simulink model "LV_Distribution"  (R2026b)
settings: Solver=VariableStepAuto
undefined symbols (not defined in the file or in its folder): P, Ts
libraries: nesl_utility x18, fl_lib x13, ee_lib x8, simulink x5, eeGeneralControl x1
settings Model: Creator=aomar  LastModifiedBy=aomar

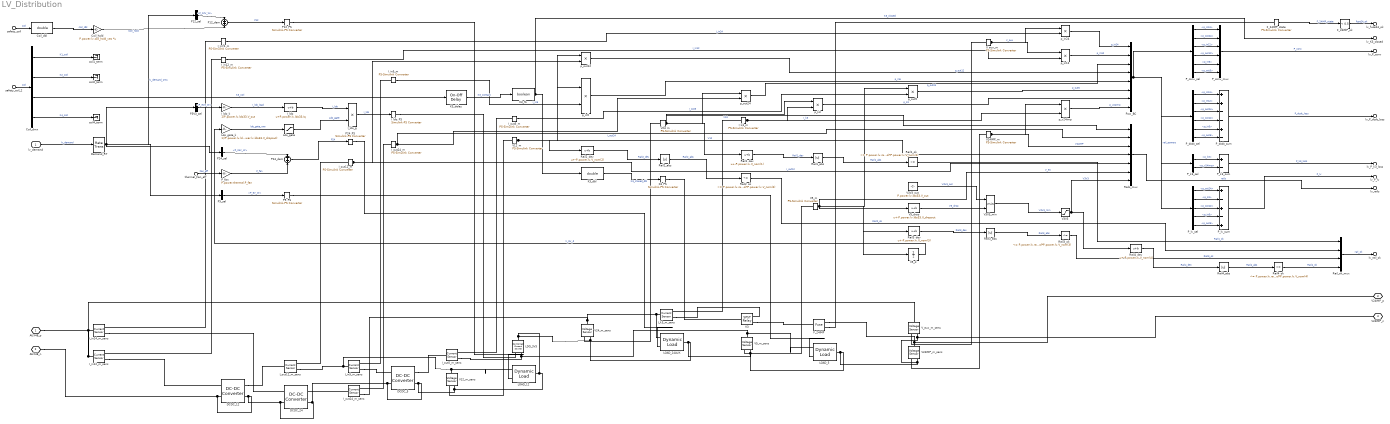
== system LV_Distribution ==
  lv_demand : Inport  OutDataTypeStr=Bus: Bus_LV_LoadDemand  SampleTime=Ts.ctrl
  thermal_Fan_eff : Inport  Port=2  PortName=thermal  Element=Fan_eff
  safety_coil : Inport  Port=3  PortName=safety  Element=coil
  safety_coil_2 : Inport  Port=3  PortName=safety  Element=coil
  Coil_dbl : DataTypeConversion  OutDataTypeStr=double  SaturateOnIntegerOverflow=off  RndMeth=Floor
  Coil_dmx : Demux
  Coil_hold : Gain  Gain=P.power.lv.coil_hold_vec  Multiplication=Matrix(K*u)
  DCDC_12 : ee_lib/Semiconductors & Converters/Converters/DC-DC Converter  Vref_option=ee.enum.converters.voltageref.internal  v_ref=P.power.lv.dcdc12.v_ref V  P_rated=P.power.lv.dcdc12.P_rated W  droop_enabled=false  droop_param=ee.enum.converters.droop.value  droop=0.1 V/A  droop_percent=2  Vref_droop=10 V  reversible=ee.enum.converters.directionality.unidirectional  G_diode=1e-8 1/Ohm  P_fixed=P.power.lv.dcdc12.P_fixed W  losses_option=ee.enum.converters.lossesOption.proportionalToSquaredCurrent  eff_rated=P.power.lv.dcdc12.eff_rated  tableOption=ee.enum.converters.lossTableOptionThermal.currentTemp  i_eff_vec=[-2, -1, 1, 2] A  v_eff_vec=[15, 30, 45] V  eff_vec=[66, 76, 80, 74]  eff_2D_table=[66, 66, 66; 76, 76, 76; 80, 80, 80; 74, 74, 74]  model_dynamics=ee.enum.converters.dynamics.yes  tau=P.power.lv.dcdc12.tau s  v_ini=0 V  v1_min=P.power.lv.dcdc12.v1_min V  R1=P.power.lv.dcdc12.R1 Ohm  R2=P.power.lv.dcdc12.R2 Ohm  T_eff_vec=[280, 300, 320] K  eff_3D_table=repmat([66; 76; 80; 74], 1, 3, 3)  thermal_mass=100 J/K  initial_temperature=298.15 K
  DCDC_24 : ee_lib/Semiconductors & Converters/Converters/DC-DC Converter  Vref_option=ee.enum.converters.voltageref.internal  v_ref=P.power.lv.dcdc24.v_ref V  P_rated=P.power.lv.dcdc24.P_rated W  droop_enabled=false  droop_param=ee.enum.converters.droop.value  droop=0.1 V/A  droop_percent=2  Vref_droop=10 V  reversible=ee.enum.converters.directionality.unidirectional  G_diode=1e-8 1/Ohm  P_fixed=P.power.lv.dcdc24.P_fixed W  losses_option=ee.enum.converters.lossesOption.proportionalToSquaredCurrent  eff_rated=P.power.lv.dcdc24.eff_rated  tableOption=ee.enum.converters.lossTableOptionThermal.currentTemp  i_eff_vec=[-2, -1, 1, 2] A  v_eff_vec=[15, 30, 45] V  eff_vec=[66, 76, 80, 74]  eff_2D_table=[66, 66, 66; 76, 76, 76; 80, 80, 80; 74, 74, 74]  model_dynamics=ee.enum.converters.dynamics.yes  tau=P.power.lv.dcdc24.tau s  v_ini=0 V  v1_min=P.power.lv.dcdc24.v1_min V  R1=P.power.lv.dcdc24.R1 Ohm  R2=P.power.lv.dcdc24.R2 Ohm  T_eff_vec=[280, 300, 320] K  eff_3D_table=repmat([66; 76; 80; 74], 1, 3, 3)  thermal_mass=100 J/K  initial_temperature=298.15 K
  DCDC_5 : ee_lib/Semiconductors & Converters/Converters/DC-DC Converter  Vref_option=ee.enum.converters.voltageref.internal  v_ref=P.power.lv.dcdc5.v_ref V  P_rated=P.power.lv.dcdc5.P_rated W  droop_enabled=false  droop_param=ee.enum.converters.droop.value  droop=0.1 V/A  droop_percent=2  Vref_droop=10 V  reversible=ee.enum.converters.directionality.unidirectional  G_diode=1e-8 1/Ohm  P_fixed=P.power.lv.dcdc5.P_fixed W  losses_option=ee.enum.converters.lossesOption.proportionalToSquaredCurrent  eff_rated=P.power.lv.dcdc5.eff_rated  tableOption=ee.enum.converters.lossTableOptionThermal.currentTemp  i_eff_vec=[-2, -1, 1, 2] A  v_eff_vec=[15, 30, 45] V  eff_vec=[66, 76, 80, 74]  eff_2D_table=[66, 66, 66; 76, 76, 76; 80, 80, 80; 74, 74, 74]  model_dynamics=ee.enum.converters.dynamics.yes  tau=P.power.lv.dcdc5.tau s  v_ini=0 V  v1_min=P.power.lv.dcdc5.v1_min V  R1=P.power.lv.dcdc5.R1 Ohm  R2=P.power.lv.dcdc5.R2 Ohm  T_eff_vec=[280, 300, 320] K  eff_3D_table=repmat([66; 76; 80; 74], 1, 3, 3)  thermal_mass=100 J/K  initial_temperature=298.15 K
  Demand_RT : RateTransition  OutPortSampleTime=Ts.base
  F_24IMP : ee_lib/Switches & Breakers/Fuse  prm=3  I_rated=1 A  melt_margin=1  T_fuse=0 s  I2t=1 A^2*s  I_vec=P.power.pdu.F_24IMP.I_vec A  t_vec=P.power.pdu.F_24IMP.t_vec s  R_closed=P.power.pdu.F_24IMP.R_closed Ohm  G_open=P.power.pdu.F_24IMP.G_open 1/Ohm  exposemeasurement=ee.enum.exposemeasurement.visible
  F_24IMP_ok : simulink/Logic and Bit Operations/Compare To Constant  relop=<  const=0.5  OutDataTypeStr=boolean
  F_24IMP_state : nesl_utility/PS-Simulink Converter  PhysicalDomain=network_engine_domain  SubClassName=ps_output  LeftPortType=input  RightPortType=output  PseudoPeriodic=off  Frequencies=[]  VectorFormat=inherit  Unit=1  AffineConversion=off
  I_in12_m : nesl_utility/PS-Simulink Converter  PhysicalDomain=network_engine_domain  SubClassName=ps_output  LeftPortType=input  RightPortType=output  PseudoPeriodic=off  Frequencies=[]  VectorFormat=inherit  Unit=A  AffineConversion=off
  I_in12_m_sens : fl_lib/Electrical/Electrical Sensors/Current Sensor
  I_in24_m : nesl_utility/PS-Simulink Converter  PhysicalDomain=network_engine_domain  SubClassName=ps_output  LeftPortType=input  RightPortType=output  PseudoPeriodic=off  Frequencies=[]  VectorFormat=inherit  Unit=A  AffineConversion=off
  I_in24_m_sens : fl_lib/Electrical/Electrical Sensors/Current Sensor
  I_in5_m : nesl_utility/PS-Simulink Converter  PhysicalDomain=network_engine_domain  SubClassName=ps_output  LeftPortType=input  RightPortType=output  PseudoPeriodic=off  Frequencies=[]  VectorFormat=inherit  Unit=A  AffineConversion=off
  I_in5_m_sens : fl_lib/Electrical/Electrical Sensors/Current Sensor
  I_k3_m : nesl_utility/PS-Simulink Converter  PhysicalDomain=network_engine_domain  SubClassName=ps_output  LeftPortType=input  RightPortType=output  PseudoPeriodic=off  Frequencies=[]  VectorFormat=inherit  Unit=A  AffineConversion=off
  I_k3_m_sens : fl_lib/Electrical/Electrical Sensors/Current Sensor
  I_ldo : Bias  Bias=P.power.lv.ldo33.Iq  SaturateOnIntegerOverflow=off
  I_ldo_PS : nesl_utility/Simulink-PS Converter  PhysicalDomain=network_engine_domain  SubClassName=ps_input  LeftPortType=input  RightPortType=output  PseudoPeriodic=off  Frequencies=[]  NoiseDistribution=none  NoiseParameters=[]  Unit=A  AffineConversion=off  FilteringAndDerivatives=zero  SimscapeFilterOrder=1  InputFilterTimeConstant=0.001  UdotUserProvided=0
  I_ldo_g : Product
  I_ldo_k : Gain  Gain=1/P.power.lv.ldo33.V_out
  I_out12_m : nesl_utility/PS-Simulink Converter  PhysicalDomain=network_engine_domain  SubClassName=ps_output  LeftPortType=input  RightPortType=output  PseudoPeriodic=off  Frequencies=[]  VectorFormat=inherit  Unit=A  AffineConversion=off
  I_out12_m_sens : fl_lib/Electrical/Electrical Sensors/Current Sensor
  I_out24_m : nesl_utility/PS-Simulink Converter  PhysicalDomain=network_engine_domain  SubClassName=ps_output  LeftPortType=input  RightPortType=output  PseudoPeriodic=off  Frequencies=[]  VectorFormat=inherit  Unit=A  AffineConversion=off
  I_out24_m_sens : fl_lib/Electrical/Electrical Sensors/Current Sensor
  I_out5_m : nesl_utility/PS-Simulink Converter  PhysicalDomain=network_engine_domain  SubClassName=ps_output  LeftPortType=input  RightPortType=output  PseudoPeriodic=off  Frequencies=[]  VectorFormat=inherit  Unit=A  AffineConversion=off
  I_out5_m_sens : fl_lib/Electrical/Electrical Sensors/Current Sensor
  K3 : ee_lib/Switches & Breakers/Relays/SPST Relay  block_choices=ee.enum.controlport.ps  R_closed=P.power.pdu.K3.R_closed Ohm  G_open=P.power.pdu.K3.G_open 1/Ohm  Threshold=0.5  exposemeasurement=ee.enum.exposemeasurement.hidden  V_rated=5 V  V_energize=75  V_deenergize=25  l_winding=0.08 H  r_winding=12.5 Ohm  g_winding=1e-9 1/Ohm  T_brk_C_S=0 s  T_mak_C_S=0 s  fault_types=ee.enum.relays.faultTypes.winding
  K3_PS : nesl_utility/Simulink-PS Converter  PhysicalDomain=network_engine_domain  SubClassName=ps_input  LeftPortType=input  RightPortType=output  PseudoPeriodic=off  Frequencies=[]  NoiseDistribution=none  NoiseParameters=[]  Unit=1  AffineConversion=off  FilteringAndDerivatives=zero  SimscapeFilterOrder=1  InputFilterTimeConstant=0.001  UdotUserProvided=0
  K3_dbl : DataTypeConversion  OutDataTypeStr=double  SaturateOnIntegerOverflow=off  RndMeth=Floor
  K3_delay : eeGeneralControl/On-Off Delay  LabelModeActiveChoice=Discrete  Td_on=P.power.pdu.K3.t_on  Td_off=P.power.pdu.K3.t_off  IC=0  Ts=Ts.base
      settings: LibrarySourceBlock=ee_sl_lib/General Control/On-Off Delay
  K3_fb : DataTypeConversion  OutDataTypeStr=boolean  RndMeth=Nearest
  LDO_3V3 : fl_lib/Electrical/Electrical Sources/Controlled Current Source
  LOAD_12 : ee_lib/Passive/Dynamic Load  load_type=ee.enum.dc_ac.dc  min_supply_voltage=P.power.lv.load.min_supply_frac*12 V  pow_min=P.power.lv.load.pow_min W  G_reverse=P.power.lv.load.G_reverse S  deltaV=P.power.lv.load.deltaV V  f0=60 Hz  Vrms_min=200 V  tau=0.01 s  Vrms_ini=300 V  Vang_ini=0 deg
  LOAD_24AUX : ee_lib/Passive/Dynamic Load  load_type=ee.enum.dc_ac.dc  min_supply_voltage=P.power.lv.load.min_supply_frac*24 V  pow_min=P.power.lv.load.pow_min W  G_reverse=P.power.lv.load.G_reverse S  deltaV=P.power.lv.load.deltaV V  f0=60 Hz  Vrms_min=200 V  tau=0.01 s  Vrms_ini=300 V  Vang_ini=0 deg
  LOAD_5 : ee_lib/Passive/Dynamic Load  load_type=ee.enum.dc_ac.dc  min_supply_voltage=P.power.lv.load.min_supply_frac*5 V  pow_min=P.power.lv.load.pow_min W  G_reverse=P.power.lv.load.G_reverse S  deltaV=P.power.lv.load.deltaV V  f0=60 Hz  Vrms_min=200 V  tau=0.01 s  Vrms_ini=300 V  Vang_ini=0 deg
  Ldo_gate : Saturate  UpperLimit=1  LowerLimit=0
  Ldo_gate_k : Gain  Gain=1/(P.power.lv.ldo33.V_out + P.power.lv.ldo33.V_dropout)
  P12_PS : nesl_utility/Simulink-PS Converter  PhysicalDomain=network_engine_domain  SubClassName=ps_input  LeftPortType=input  RightPortType=output  PseudoPeriodic=off  Frequencies=[]  NoiseDistribution=none  NoiseParameters=[]  Unit=W  AffineConversion=off  FilteringAndDerivatives=zero  SimscapeFilterOrder=1  InputFilterTimeConstant=0.001  UdotUserProvided=0
  P12_dem : Sum
  P12_sel : BusSelector  OutputSignals=P_12V_W
  P24_PS : nesl_utility/Simulink-PS Converter  PhysicalDomain=network_engine_domain  SubClassName=ps_input  LeftPortType=input  RightPortType=output  PseudoPeriodic=off  Frequencies=[]  NoiseDistribution=none  NoiseParameters=[]  Unit=W  AffineConversion=off  FilteringAndDerivatives=zero  SimscapeFilterOrder=1  InputFilterTimeConstant=0.001  UdotUserProvided=0
  P24_dem : Sum
  P24_sel : BusSelector  OutputSignals=P_24V_W
  P3V3_sel : BusSelector  OutputSignals=P_3V3_W
  P5_PS : nesl_utility/Simulink-PS Converter  PhysicalDomain=network_engine_domain  SubClassName=ps_input  LeftPortType=input  RightPortType=output  PseudoPeriodic=off  Frequencies=[]  NoiseDistribution=none  NoiseParameters=[]  Unit=W  AffineConversion=off  FilteringAndDerivatives=zero  SimscapeFilterOrder=1  InputFilterTimeConstant=0.001  UdotUserProvided=0
  P5_sel : BusSelector  OutputSignals=P_5V_W
  P_conv_mux : Mux  Inputs=6
  P_conv_sel : BusSelector  OutputSignals=p_in24,p_out24,p_in12,p_out12,p_in5,p_out5
  P_dcdc_sel : BusSelector  OutputSignals=p_in24,p_in12,p_out24,p_out12,p_in5,p_out5
  P_dcdc_sum : Sum  Inputs=++--+-
  P_fan : Gain  Gain=P.power.thermal.P_fan
  P_k3_sel : BusSelector  OutputSignals=p_k3,p_v24imp
  P_k3_sum : Sum  Inputs=+-
  P_lv_sel : BusSelector  OutputSignals=p_out24,p_k3,p_out12,p_in5,p_out5
  P_lv_sum : Sum  Inputs=+-+-+
  Pow_BC : BusCreator  Inputs=8
  Rail1_abs : Abs  SaturateOnIntegerOverflow=off
  Rail1_dev : Bias  Bias=-P.power.lv.V_nom(1)  SaturateOnIntegerOverflow=off
  Rail1_ok : simulink/Logic and Bit Operations/Compare To Constant  relop=<=  const=P.power.lv.rail_ok_tol*P.power.lv.V_nom(1)  OutDataTypeStr=boolean
  Rail2_abs : Abs  SaturateOnIntegerOverflow=off
  Rail2_dev : Bias  Bias=-P.power.lv.V_nom(2)  SaturateOnIntegerOverflow=off
  Rail2_ok : simulink/Logic and Bit Operations/Compare To Constant  relop=<=  const=P.power.lv.rail_ok_tol*P.power.lv.V_nom(2)  OutDataTypeStr=boolean
  Rail3_abs : Abs  SaturateOnIntegerOverflow=off
  Rail3_dev : Bias  Bias=-P.power.lv.V_nom(3)  SaturateOnIntegerOverflow=off
  Rail3_ok : simulink/Logic and Bit Operations/Compare To Constant  relop=<=  const=P.power.lv.rail_ok_tol*P.power.lv.V_nom(3)  OutDataTypeStr=boolean
  Rail4_abs : Abs  SaturateOnIntegerOverflow=off
  Rail4_dev : Bias  Bias=-P.power.lv.V_nom(4)  SaturateOnIntegerOverflow=off
  Rail4_ok : simulink/Logic and Bit Operations/Compare To Constant  relop=<=  const=P.power.lv.rail_ok_tol*P.power.lv.V_nom(4)  OutDataTypeStr=boolean
  Rail_ok_mux : Mux
  Rails_mux : Mux  Inputs=7
  V12_m : nesl_utility/PS-Simulink Converter  PhysicalDomain=network_engine_domain  SubClassName=ps_output  LeftPortType=input  RightPortType=output  PseudoPeriodic=off  Frequencies=[]  VectorFormat=inherit  Unit=V  AffineConversion=off
  V12_m_sens : fl_lib/Electrical/Electrical Sensors/Voltage Sensor
  V24IMP_m : nesl_utility/PS-Simulink Converter  PhysicalDomain=network_engine_domain  SubClassName=ps_output  LeftPortType=input  RightPortType=output  PseudoPeriodic=off  Frequencies=[]  VectorFormat=inherit  Unit=V  AffineConversion=off
  V24IMP_m_sens : fl_lib/Electrical/Electrical Sensors/Voltage Sensor
  V24_m : nesl_utility/PS-Simulink Converter  PhysicalDomain=network_engine_domain  SubClassName=ps_output  LeftPortType=input  RightPortType=output  PseudoPeriodic=off  Frequencies=[]  VectorFormat=inherit  Unit=V  AffineConversion=off
  V24_m_sens : fl_lib/Electrical/Electrical Sensors/Voltage Sensor
  V3V3 : Saturate  UpperLimit=inf  LowerLimit=0
  V3V3_min : MinMax  Inputs=2
  V3V3_out : Constant  Value=P.power.lv.ldo33.V_out  SampleTime=Ts.base
  V5_d : UnitDelay  SampleTime=Ts.base
  V5_drop : Bias  Bias=-P.power.lv.ldo33.V_dropout  SaturateOnIntegerOverflow=off
  V5_m : nesl_utility/PS-Simulink Converter  PhysicalDomain=network_engine_domain  SubClassName=ps_output  LeftPortType=input  RightPortType=output  PseudoPeriodic=off  Frequencies=[]  VectorFormat=inherit  Unit=V  AffineConversion=off
  V5_m_sens : fl_lib/Electrical/Electrical Sensors/Voltage Sensor
  V_aux_m : nesl_utility/PS-Simulink Converter  PhysicalDomain=network_engine_domain  SubClassName=ps_output  LeftPortType=input  RightPortType=output  PseudoPeriodic=off  Frequencies=[]  VectorFormat=inherit  Unit=V  AffineConversion=off
  V_aux_m_sens : fl_lib/Electrical/Electrical Sensors/Voltage Sensor
  coil1_term : Terminator
  coil2_term : Terminator
  coil4_term : Terminator
  p_in12 : Product
  p_in24 : Product
  p_in5 : Product
  p_k3 : Product
  p_out12 : Product
  p_out24 : Product
  p_out5 : Product
  p_v24imp : Product
  AUX48_p : PMIOPort  Side=Left  ConnectionType=Connection: foundation.electrical.electrical
  AUX48_n : PMIOPort  Port=2  Side=Left  ConnectionType=Connection: foundation.electrical.electrical
  V24IMP_p : PMIOPort  Port=3  Side=Right  ConnectionType=Connection: foundation.electrical.electrical
  V24IMP_n : PMIOPort  Port=4  Side=Right  ConnectionType=Connection: foundation.electrical.electrical
  lv_rails : Outport  PortName=lv  Element=rails
  lv_rail_ok : Outport  PortName=lv  Element=rail_ok
  lv_K3_closed : Outport  PortName=lv  Element=K3_closed
  lv_fuse24_ok : Outport  PortName=lv  Element=fuse24_ok
  lv_P_lv : Outport  PortName=lv  Element=P_lv
  lv_P_dcdc_loss : Outport  PortName=lv  Element=P_dcdc_loss
  lv_P_k3_loss : Outport  PortName=lv  Element=P_k3_loss
  lv_P_conv : Outport  PortName=lv  Element=P_conv
  wires:
  safety_coil/1 -> Coil_dbl/1  "coil"
  safety_coil_2/1 -> Coil_dmx/1  "coil"
  Coil_dmx/1 -> coil1_term/1  "K1_coil"
  Coil_dmx/2 -> coil2_term/1  "K2_coil"
  Coil_dmx/3 -> K3_delay/1  "K3_coil"
  Coil_dmx/4 -> coil4_term/1  "K4_coil"
  lv_demand/1 -> Demand_RT/1  "lv_demand"
  Coil_dbl/1 -> Coil_hold/1  "coil_dbl"
  Coil_hold/1 -> P12_dem/2  "Coil_hold"
  Demand_RT/1 -> P12_sel/1, P5_sel/1, P3V3_sel/1, P24_sel/1  "lv_demand_1ms"
  P12_sel/1 -> P12_dem/1  "<P_12V_W>"
  P3V3_sel/1 -> I_ldo_k/1  "<P_3V3_W>"
  thermal_Fan_eff/1 -> P_fan/1  "Fan_eff"
  P24_sel/1 -> P24_dem/1  "<P_24V_W>"
  P5_sel/1 -> P5_PS/1  "<P_5V_W>"
  I_in24_m/1 -> p_in24/2  "I_in24"
  I_in12_m/1 -> p_in12/2  "I_in12"
  P12_dem/1 -> P12_PS/1  "P12"
  I_ldo_k/1 -> I_ldo/1  "I_ldo_load"
  Ldo_gate_k/1 -> Ldo_gate/1  "ldo_gate_raw"
  P_fan/1 -> P24_dem/2  "P_fan"
  P24_dem/1 -> P24_PS/1  "P24"
  Ldo_gate/1 -> I_ldo_g/2  "Ldo_gate"
  I_ldo/1 -> I_ldo_g/1  "I_ldo"
  I_out12_m/1 -> p_out12/2, Rails_mux/5  "I_out12"
  I_ldo_g/1 -> I_ldo_PS/1  "I_ldo"
  I_in5_m/1 -> p_in5/2  "I_in5"
  I_out24_m/1 -> p_out24/2, Rails_mux/2  "I_out24"
  K3_delay/1 -> K3_fb/1  "K3_contact"
  I_out5_m/1 -> p_out5/2  "I_out5"
  V12_m/1 -> p_out12/1, p_in5/1, Rails_mux/4, Rail2_dev/1  "V12"
  K3_fb/1 -> K3_dbl/1, lv_K3_closed/1  "K3_closed"
  p_out12/1 -> Pow_BC/4  "p_out12"
  p_in5/1 -> Pow_BC/5  "p_in5"
  Rail2_dev/1 -> Rail2_abs/1  "Rail2_dev"
  K3_dbl/1 -> K3_PS/1  "K3_closed_dbl"
  V24_m/1 -> Rail1_dev/1, p_out24/1, p_k3/1, Rails_mux/1  "V24"
  Rail2_abs/1 -> Rail2_ok/1  "Rail2_abs"
  I_k3_m/1 -> p_k3/2, p_v24imp/2  "I_k3"
  p_out24/1 -> Pow_BC/3  "p_out24"
  Rail2_ok/1 -> Rail_ok_mux/2  "Rail2_ok"
  Rail1_dev/1 -> Rail1_abs/1  "Rail1_dev"
  V5_m/1 -> p_out5/1, V5_d/1, Rails_mux/6, Rail3_dev/1, V5_drop/1  "V_5V"
  p_k3/1 -> Pow_BC/7  "p_k3"
  Rail1_abs/1 -> Rail1_ok/1  "Rail1_abs"
  p_out5/1 -> Pow_BC/6  "p_out5"
  Rail1_ok/1 -> Rail_ok_mux/1  "Rail1_ok"
  V3V3_out/1 -> V3V3_min/1  "V3V3_out"
  V5_d/1 -> Ldo_gate_k/1  "V_5V_d"
  V5_drop/1 -> V3V3_min/2  "V5_drop"
  Rail3_dev/1 -> Rail3_abs/1  "Rail3_dev"
  V_aux_m/1 -> p_in24/1, p_in12/1  "V_aux"
  V24IMP_m/1 -> p_v24imp/1, Rails_mux/3  "V24IMP"
  V3V3_min/1 -> V3V3/1  "V3V3_min"
  Rail3_abs/1 -> Rail3_ok/1  "Rail3_abs"
  p_in24/1 -> Pow_BC/1  "p_in24"
  p_in12/1 -> Pow_BC/2  "p_in12"
  p_v24imp/1 -> Pow_BC/8  "p_v24imp"
  V3V3/1 -> Rail4_dev/1, Rails_mux/7  "V3V3"
  Rail3_ok/1 -> Rail_ok_mux/3  "Rail3_ok"
  Pow_BC/1 -> P_lv_sel/1, P_k3_sel/1, P_dcdc_sel/1, P_conv_sel/1  "rail_powers"
  Rails_mux/1 -> lv_rails/1  "rails"
  Rail4_dev/1 -> Rail4_abs/1  "Rail4_dev"
  P_conv_sel/1 -> P_conv_mux/1  "<p_in24>"
  P_conv_sel/2 -> P_conv_mux/2  "<p_out24>"
  P_conv_sel/3 -> P_conv_mux/3  "<p_in12>"
  P_conv_sel/4 -> P_conv_mux/4  "<p_out12>"
  P_conv_sel/5 -> P_conv_mux/5  "<p_in5>"
  P_conv_sel/6 -> P_conv_mux/6  "<p_out5>"
  P_dcdc_sel/1 -> P_dcdc_sum/1  "<p_in24>"
  P_dcdc_sel/2 -> P_dcdc_sum/2  "<p_in12>"
  P_dcdc_sel/3 -> P_dcdc_sum/3  "<p_out24>"
  P_dcdc_sel/4 -> P_dcdc_sum/4  "<p_out12>"
  P_dcdc_sel/5 -> P_dcdc_sum/5  "<p_in5>"
  P_dcdc_sel/6 -> P_dcdc_sum/6  "<p_out5>"
  P_k3_sel/1 -> P_k3_sum/1  "<p_k3>"
  P_k3_sel/2 -> P_k3_sum/2  "<p_v24imp>"
  P_lv_sel/1 -> P_lv_sum/1  "<p_out24>"
  P_lv_sel/2 -> P_lv_sum/2  "<p_k3>"
  P_lv_sel/3 -> P_lv_sum/3  "<p_out12>"
  P_lv_sel/4 -> P_lv_sum/4  "<p_in5>"
  P_lv_sel/5 -> P_lv_sum/5  "<p_out5>"
  P_conv_mux/1 -> lv_P_conv/1  "P_conv"
  P_dcdc_sum/1 -> lv_P_dcdc_loss/1  "P_dcdc_loss"
  P_k3_sum/1 -> lv_P_k3_loss/1  "P_k3_loss"
  P_lv_sum/1 -> lv_P_lv/1  "P_lv"
  Rail4_abs/1 -> Rail4_ok/1  "Rail4_abs"
  F_24IMP_state/1 -> F_24IMP_ok/1  "F_24IMP_state"
  Rail4_ok/1 -> Rail_ok_mux/4  "Rail4_ok"
  Rail_ok_mux/1 -> lv_rail_ok/1  "rail_ok"
  F_24IMP_ok/1 -> lv_fuse24_ok/1  "fuse24_ok"
  connections:
  DCDC_12/LConn2 -- AUX48_n/RConn1 -- DCDC_12/RConn2 -- DCDC_24/LConn2 -- DCDC_24/RConn2 -- DCDC_5/LConn2 -- DCDC_5/RConn2 -- V12_m_sens/RConn2 -- LOAD_12/RConn1 -- LDO_3V3/LConn1 -- V24_m_sens/RConn2 -- LOAD_24AUX/RConn1 -- V5_m_sens/RConn2 -- LOAD_5/RConn1 -- V24IMP_m_sens/RConn2 -- V_aux_m_sens/RConn2 -- V24IMP_n/RConn1
  I_in24_m_sens/LConn1 -- AUX48_p/RConn1 -- I_in12_m_sens/LConn1 -- V_aux_m_sens/LConn1
  I_in12_m_sens/RConn2 -- DCDC_12/LConn1
  DCDC_12/RConn1 -- I_out12_m_sens/LConn1
  I_in24_m_sens/RConn2 -- DCDC_24/LConn1
  DCDC_24/RConn1 -- I_out24_m_sens/LConn1
  I_in5_m_sens/RConn2 -- DCDC_5/LConn1
  DCDC_5/RConn1 -- I_out5_m_sens/LConn1
  K3/RConn2 -- F_24IMP/LConn1
  V24IMP_m_sens/LConn1 -- F_24IMP/RConn1 -- V24IMP_p/RConn1
  F_24IMP/RConn2 -- F_24IMP_state/LConn1
  I_in12_m/LConn1 -- I_in12_m_sens/RConn1
  I_in24_m/LConn1 -- I_in24_m_sens/RConn1
  I_in5_m/LConn1 -- I_in5_m_sens/RConn1
  I_in5_m_sens/LConn1 -- I_out12_m_sens/RConn2 -- V12_m_sens/LConn1 -- LOAD_12/LConn1
  I_k3_m/LConn1 -- I_k3_m_sens/RConn1
  V24_m_sens/LConn1 -- I_out24_m_sens/RConn2 -- I_k3_m_sens/LConn1 -- LOAD_24AUX/LConn1
  I_k3_m_sens/RConn2 -- K3/RConn1
  I_ldo_PS/RConn1 -- LDO_3V3/RConn1
  I_out12_m/LConn1 -- I_out12_m_sens/RConn1
  I_out24_m/LConn1 -- I_out24_m_sens/RConn1
  I_out5_m/LConn1 -- I_out5_m_sens/RConn1
  LDO_3V3/RConn2 -- I_out5_m_sens/RConn2 -- V5_m_sens/LConn1 -- LOAD_5/LConn1
  K3_PS/RConn1 -- K3/LConn1
  P12_PS/RConn1 -- LOAD_12/LConn2
  P24_PS/RConn1 -- LOAD_24AUX/LConn2
  P5_PS/RConn1 -- LOAD_5/LConn2
  V12_m/LConn1 -- V12_m_sens/RConn1
  V24IMP_m/LConn1 -- V24IMP_m_sens/RConn1
  V24_m/LConn1 -- V24_m_sens/RConn1
  V5_m/LConn1 -- V5_m_sens/RConn1
  V_aux_m/LConn1 -- V_aux_m_sens/RConn1
